simulink model "schemat"  (R2025b)
settings: Solver=ode1  StartTime=0.0  StopTime=10.0  FixedStep=Ts/10  RelTol=1e-3
values from neighbouring files (symbols this model uses):
  K = 2.0    (= 2)    [init.m]
  Kd = Kp * Td    [init.m]
  Ki = Kp / Ti    [init.m]
  Kp = (1.2 * Tz) / (K * L)    [init.m]
  r = r_vec(r_idx)    [ZN.m]
  Ta = 3.0    (= 3)    [init.m]
  tau = tau_vec(t_idx)    [ZN.m]    (also in init.m = 0)
  Tb = 2.0    (= 2)    [init.m]
  Ts = 0.05    [init.m]
  Umax = umax_vec(u_idx)    [ZN.m]    (also in init.m = 3)
  Umin = 0.0    (= 0)    [init.m]
  y0 = 1.0    (= 1)    [init.m]
libraries: slpidlib x1
settings Model: Creator=Karolina  LastModifiedBy=Karolina

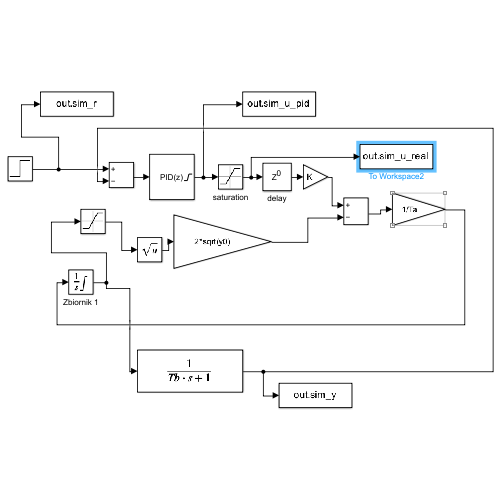
[thumbnail: Simulink's stored preview of the top-level diagram]
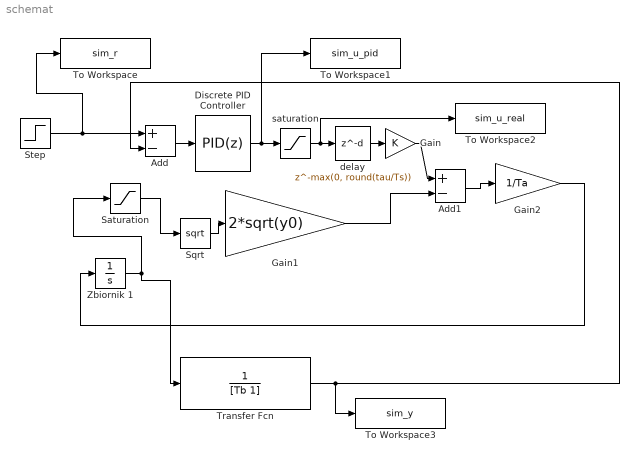
== system schemat ==
  Add : Sum  Inputs=+-
  Add1 : Sum  Inputs=+-
  Discrete PID Controller : slpidlib/PID Controller  Controller=PID  Form=Parallel  TimeDomain=Discrete-time  UseExternalTs=off  SampleTime=Ts  IntegratorMethod=Forward Euler  FilterMethod=Backward Euler  ControllerParametersSource=internal  P=Kp  I=Ki  UseKiTs=off  D=Kd  UseExternalDerivativeSource=off  N=100  UseFilter=on  TunerSelectOption=Transfer Function Based (PID Tuner App)  InitialConditionSource=internal  InitialConditionForIntegrator=0  InitialConditionForFilter=0  DifferentiatorICPrevScaledInput=0  ExternalReset=none  TrackingMode=off  Kt=1  LimitOutput=on  SatLimitsSource=internal  UpperSaturationLimit=Umax  LowerSaturationLimit=Umin  LinearizeAsGain=off  AntiWindupMode=clamping  Kb=1  LimitIntegrator=off  UpperIntegratorSaturationLimit=Umax  LowerIntegratorSaturationLimit=Umin  RndMeth=Ceiling  POutMin=[]  POutMax=[]  IOutMin=[]  IOutMax=[]  DOutMin=[]  DOutMax=[]  NOutMin=[]  NOutMax=[]  SumOutMin=[]  SumOutMax=[]  SaturationOutMin=[]  SaturationOutMax=[]  PParamMin=[]  PParamMax=[]  IParamMin=[]  IParamMax=[]  DParamMin=[]  DParamMax=[]  NParamMin=[]  NParamMax=[]  KbParamMin=[]  KbParamMax=[]  KtParamMin=[]  KtParamMax=[]  KbOutMin=[]  KbOutMax=[]  KtOutMin=[]  KtOutMax=[]  IntegratorOutMin=[]  IntegratorOutMax=[]  FilterOutMin=[]  FilterOutMax=[]  SumI1OutMin=[]  SumI1OutMax=[]  SumI2OutMin=[]  SumI2OutMax=[]  SumI3OutMin=[]  SumI3OutMax=[]  SumI4OutMin=[]  SumI4OutMax=[]  SumDOutMin=[]  SumDOutMax=[]  DifferentiatorOutMin=[]  DifferentiatorOutMax=[]  FilterDiffOutCoefMin=[]  FilterDiffOutCoefMax=[]  ReciprocalOutMin=[]  ReciprocalOutMax=[]  SumDenOutMin=[]  SumDenOutMax=[]  SumNumOutMin=[]  SumNumOutMax=[]  DivideOutMin=[]  DivideOutMax=[]  UdiffTsProdOutMin=[]  UdiffTsProdOutMax=[]  NTsProdOutMin=[]  NTsProdOutMax=[]  UintegralTsProdOutMin=[]  UintegralTsProdOutMax=[]  UngainTsProdOutMin=[]  UngainTsProdOutMax=[]  ClampingZeroOutDataTypeStr=Inherit: Inherit via back propagation  ClampingZeroOutMin=[]  ClampingZeroOutMax=[]  FilterDenConstantOutDataTypeStr=Inherit: Inherit via back propagation  FilterDenConstantOutMin=[]  FilterDenConstantOutMax=[]  PCopyOutDataTypeStr=Inherit: Inherit via back propagation  PCopyOutMin=[]  PCopyOutMax=[]  NCopyOutDataTypeStr=Inherit: Inherit via back propagation  NCopyOutMin=[]  NCopyOutMax=[]  IntegratorContinuousStateAttributes=''  IntegratorStateMustResolveToSignalObject=off  IntegratorRTWStateStorageClass=Auto  FilterContinuousStateAttributes=''  FilterStateMustResolveToSignalObject=off  FilterRTWStateStorageClass=Auto  ParallelPVariant=InternalParameters  IdealPVariant=Disabled  IVariant=InternalParameters  DVariant=InternalParameters  IntegratorVariant=Discrete  SatVariant=Enabled  AWVariant=DiscClampingParallel  PCopyVariant=Disabled  TRVariant=Disabled  FdbkBlocksVariant=Forward  IdealPFdbkVariant=Disabled  SatFdbkVariant=Disabled  DerivativeFilterVariant=BackwardEulerFilter  NVariant=InternalParameters  NCopyVariant=InternalParameters  FilterICVariant=InternalICsFilter  IntegratorICVariant=InternalICs  ExternalResetVariant=Disabled  TRSumVariant=Passthrough  SumFdbkVariant=Disabled  SumVariant=Sum_PID  TsampFilterVariant=InternalTs  TsampNgainVariant=Passthrough  TsampIntegralVariant=Disabled_SignalSpec  ExternalSaturationOutDataTypeStr=Inherit: Same as second input  DerivativeSourceVariant=ErrorSignal  PreIntVariant=InternalPreInt
      settings: LibrarySourceBlock=simulink/Discrete/Discrete PID Controller
  Gain : Gain  Gain=K
  Gain1 : Gain  Gain=2*sqrt(y0)
  Gain2 : Gain  Gain=1/Ta
  Saturation : Saturate  UpperLimit=inf  LowerLimit=0
  Sqrt : Sqrt
  Step : Step  After=r  SampleTime=0
  To Workspace : ToWorkspace  VariableName=sim_r  SaveFormat=Timeseries  SampleTime=Ts
  To Workspace1 : ToWorkspace  VariableName=sim_u_pid  SaveFormat=Timeseries  SampleTime=Ts
  To Workspace2 : ToWorkspace  VariableName=sim_u_real  SaveFormat=Timeseries  SampleTime=Ts
  To Workspace3 : ToWorkspace  VariableName=sim_y  SaveFormat=Timeseries  SampleTime=Ts
  Transfer Fcn : TransferFcn  Denominator=[Tb 1]
  Zbiornik 1 : Integrator  InitialCondition=y0  LimitOutput=on  UpperSaturationLimit=20  LowerSaturationLimit=0
  delay : Delay  DelayLength=max(0, round(tau/Ts))  InitialCondition=0  SampleTime=Ts
  saturation : Saturate  UpperLimit=Umax  LowerLimit=Umin
  wires:
  Step/1 -> To Workspace/1, Add/1
  Add/1 -> Discrete PID Controller/1
  Discrete PID Controller/1 -> To Workspace1/1, saturation/1
  saturation/1 -> To Workspace2/1, delay/1
  delay/1 -> Gain/1
  Gain/1 -> Add1/1
  Add1/1 -> Gain2/1
  Zbiornik 1/1 -> Transfer Fcn/1, Saturation/1
  Sqrt/1 -> Gain1/1
  Gain1/1 -> Add1/2
  Transfer Fcn/1 -> To Workspace3/1, Add/2
  Gain2/1 -> Zbiornik 1/1
  Saturation/1 -> Sqrt/1
